simulink library "Libs_second"  (R2023b)
settings: Solver=VariableStepAuto  StartTime=0.0  StopTime=10.0  RelTol=1e-3
libraries: $bdroot x3, simulink x1
(part 1 of 2)
settings Model: Creator=wai484  LastModifiedBy=wai484
settings SolverCC: AlgebraicLoopSolver=TrustRegion
settings DataIOCC: ReturnWorkspaceOutputs=off
settings DebuggingCC: UnconnectedInputMsg=warning  UnconnectedOutputMsg=warning  UnconnectedLineMsg=warning  ArithmeticOperatorsInVariantConditions=warning
settings ModelReferenceCC: EnableRefExpFcnMdlSchedulingChecks=on
settings SFSimCC: SimUseLocalCustomCode=off  CustomCodeUndefinedFunction=UseInterfaceOnly
settings RTWCC: RTWUseLocalCustomCode=off
settings CodeAppCC: StateflowObjectComments=on

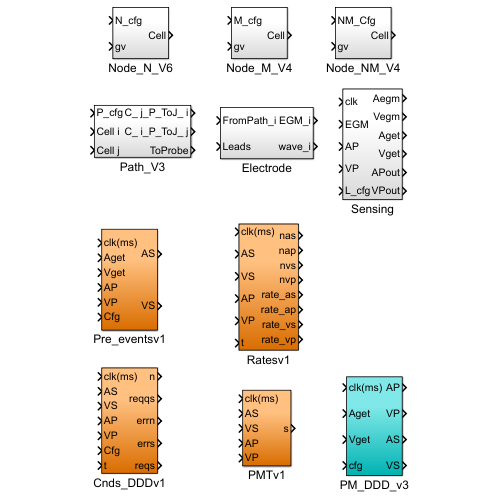
[thumbnail: Simulink's stored preview of the top-level diagram]
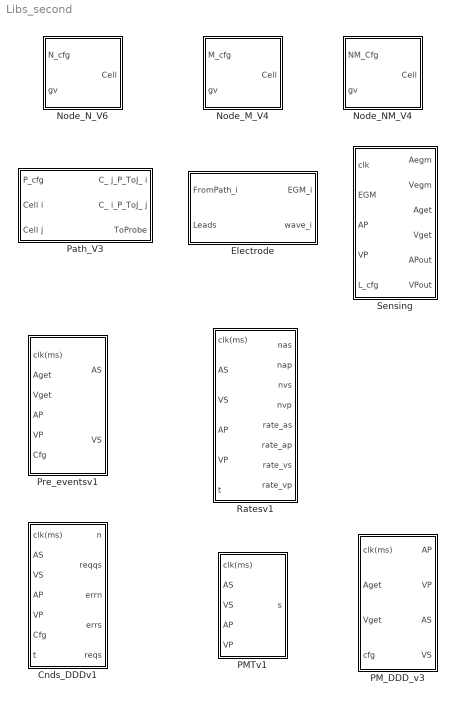
== system Libs_second ==
  Cnds_DDDv1 : Subsystem
  Electrode : Subsystem
  Node_M_V4 : Subsystem
  Node_NM_V4 : Subsystem
  Node_N_V6 : Subsystem
  PMTv1 : Subsystem
  PM_DDD_v3 : Subsystem
  Path_V3 : Subsystem
  Pre_eventsv1 : Subsystem
  Ratesv1 : Subsystem
  Sensing : Subsystem

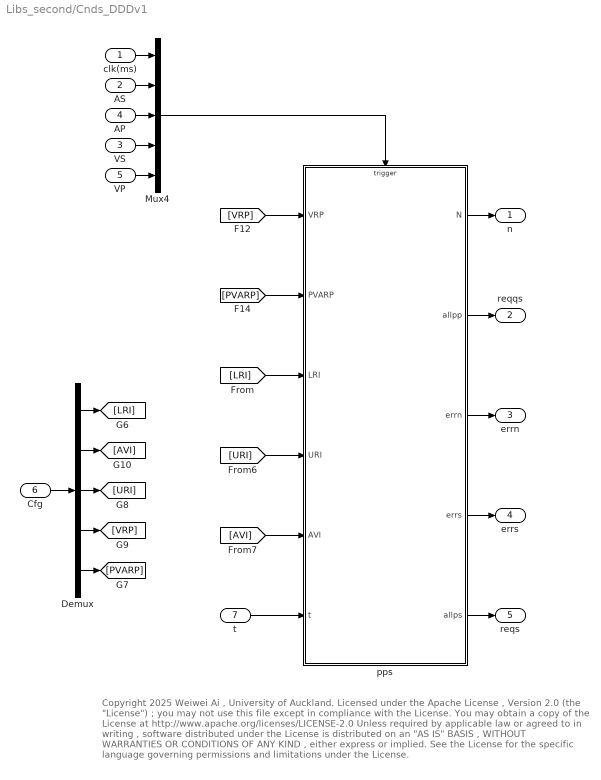
== system Libs_second/Cnds_DDDv1 ==
  note: Copyright 2025 Weiwei Ai , University of Auckland.
      | Licensed under the Apache License , Version 2.0 (the "License") ;
      | you may not use this file except in compliance with the License.
      | You may obtain a copy of the License at
      | http://www.apache.org/licenses/LICENSE-2.0
      | Unless required by applicable law or agreed to in writing , software
      | distributed under the License is distributed on an "AS IS" BASIS ,
      | WITHOUT WARRANTIES OR CONDITIONS OF ANY KIND , either express or implied.
      | See the License for the specific language governing permissions and
      | limitations under the License.
  clk(ms) : Inport
  AS : Inport  Port=2
  VS : Inport  Port=3
  AP : Inport  Port=4
  VP : Inport  Port=5
  Cfg : Inport  Port=6
  t : Inport  Port=7
  Demux : Demux  Outputs=5
  Mux4 : Mux  Inputs=5
  pps : Stateflow chart  TreatAsAtomicUnit=on
  n : Outport
  reqqs : Outport  Port=2
  errn : Outport  Port=3
  errs : Outport  Port=4
  reqs : Outport  Port=5
  wires:
  t/1 -> pps/6(t)
  pps/5(allps) -> reqs/1
  Demux/5 -> [PVARP]
  Demux/4 -> [VRP]
  Demux/3 -> [URI]
  Demux/2 -> [AVI]
  Demux/1 -> [LRI]
  pps/4(errs) -> errs/1
  pps/3(errn) -> errn/1
  pps/2(allpp) -> reqqs/1
  pps/1(N) -> n/1
  [VRP] -> pps/1(VRP)
  [PVARP] -> pps/2(PVARP)
  [LRI] -> pps/3(LRI)
  [AVI] -> pps/5(AVI)
  [URI] -> pps/4(URI)
  Cfg/1 -> Demux/1
  clk(ms)/1 -> Mux4/1
  AS/1 -> Mux4/2
  VP/1 -> Mux4/5
  Mux4/1 -> pps/Trigger
  AP/1 -> Mux4/3
  VS/1 -> Mux4/4

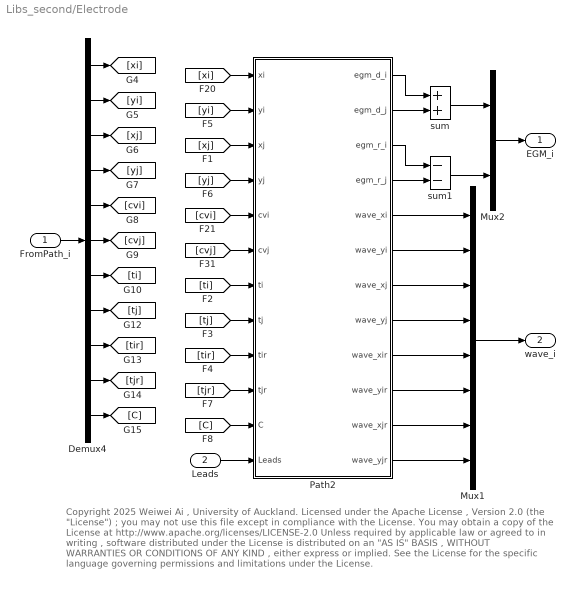
== system Libs_second/Electrode ==
  note: Copyright 2025 Weiwei Ai , University of Auckland.
      | Licensed under the Apache License , Version 2.0 (the "License") ;
      | you may not use this file except in compliance with the License.
      | You may obtain a copy of the License at
      | http://www.apache.org/licenses/LICENSE-2.0
      | Unless required by applicable law or agreed to in writing , software
      | distributed under the License is distributed on an "AS IS" BASIS ,
      | WITHOUT WARRANTIES OR CONDITIONS OF ANY KIND , either express or implied.
      | See the License for the specific language governing permissions and
      | limitations under the License.
  FromPath_i : Inport
  Leads : Inport  Port=2
  Demux4 : Demux  Outputs=11
  Mux1 : Mux  Inputs=8
  Mux2 : Mux  Inputs=2
  Path2 : Stateflow chart  TreatAsAtomicUnit=on
  sum : Sum
  sum1 : Sum  Inputs=--
  EGM_i : Outport
  wave_i : Outport  Port=2
  wires:
  Mux2/1 -> EGM_i/1
  [xi] -> Path2/1(xi)
  [xj] -> Path2/3(xj)
  [yi] -> Path2/2(yi)
  [yj] -> Path2/4(yj)
  [cvi] -> Path2/5(cvi)
  [cvj] -> Path2/6(cvj)
  FromPath_i/1 -> Demux4/1
  Demux4/1 -> [xi]
  Demux4/2 -> [yi]
  Demux4/3 -> [xj]
  Demux4/4 -> [yj]
  Demux4/5 -> [cvi]
  Demux4/6 -> [cvj]
  Demux4/7 -> [ti]
  Demux4/8 -> [tj]
  Demux4/9 -> [tir]
  Demux4/10 -> [tjr]
  Demux4/11 -> [C]
  Path2/5(wave_xi) -> Mux1/1
  Path2/6(wave_yi) -> Mux1/2
  Path2/7(wave_xj) -> Mux1/3
  Path2/8(wave_yj) -> Mux1/4
  [C] -> Path2/11(C)
  [tjr] -> Path2/10(tjr)
  [tir] -> Path2/9(tir)
  [tj] -> Path2/8(tj)
  [ti] -> Path2/7(ti)
  Leads/1 -> Path2/12(Leads)
  Path2/9(wave_xir) -> Mux1/5
  Path2/10(wave_yir) -> Mux1/6
  Path2/11(wave_xjr) -> Mux1/7
  Path2/12(wave_yjr) -> Mux1/8
  Mux1/1 -> wave_i/1
  sum/1 -> Mux2/1
  Path2/1(egm_d_i) -> sum/1
  Path2/2(egm_d_j) -> sum/2
  sum1/1 -> Mux2/2
  Path2/3(egm_r_i) -> sum1/1
  Path2/4(egm_r_j) -> sum1/2

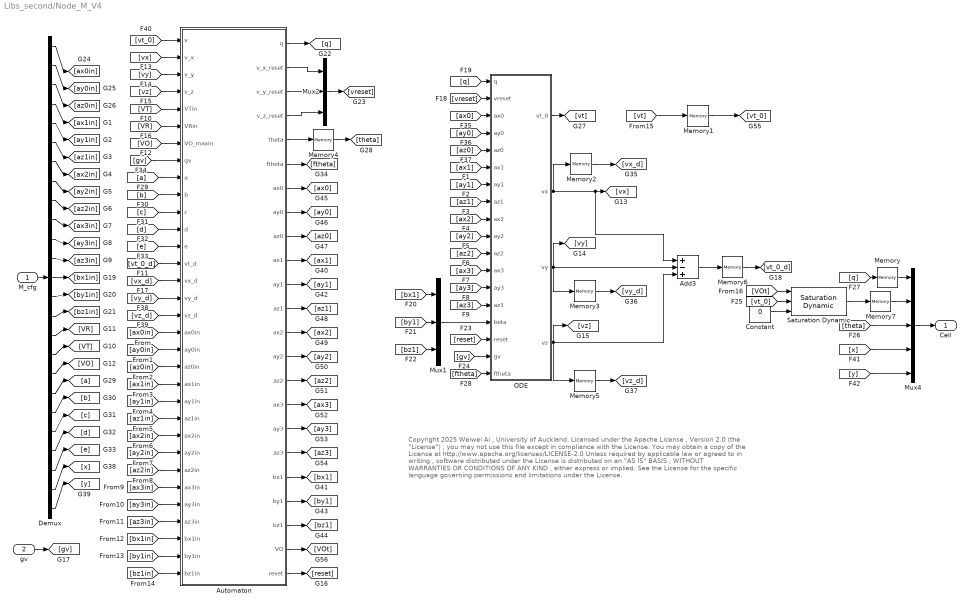
== system Libs_second/Node_M_V4 ==
  note: Copyright 2025 Weiwei Ai , University of Auckland.
      | Licensed under the Apache License , Version 2.0 (the "License") ;
      | you may not use this file except in compliance with the License.
      | You may obtain a copy of the License at
      | http://www.apache.org/licenses/LICENSE-2.0
      | Unless required by applicable law or agreed to in writing , software
      | distributed under the License is distributed on an "AS IS" BASIS ,
      | WITHOUT WARRANTIES OR CONDITIONS OF ANY KIND , either express or implied.
      | See the License for the specific language governing permissions and
      | limitations under the License.
  M_cfg : Inport
  gv : Inport  Port=2
  Add3 : Sum  Inputs=+-+
  Automaton : Stateflow chart  TreatAsAtomicUnit=on
  Constant : Constant  Value=0
  Demux : Demux  Outputs=25
  Memory : Memory
  Memory{1..3,5..7} (6 alike) : Memory  InheritSampleTime=on  LinearizeAsDelay=on
  Memory4 : Memory
  Mux1 : Mux  Inputs=3
  Mux2 : Mux  Inputs=3
  Mux4 : Mux  Inputs=5
  ODE : Subsystem
  Saturation Dynamic : simulink/Discontinuities/Saturation Dynamic  OutMin=[]  OutMax=[]  OutDataTypeStr=Inherit: Same as second input  OutDataType=fixdt(1, 16)  OutScaling=2^-10  DoSatur=off
  Cell : Outport
  wires:
  M_cfg/1 -> Demux/1
  Automaton/2(v_x_reset) -> Mux2/1
  Automaton/3(v_y_reset) -> Mux2/2
  Automaton/4(v_z_reset) -> Mux2/3
  Mux4/1 -> Cell/1
  Demux/1 -> [ax0in]
  [ax0] -> ODE/3(ax0)
  Demux/2 -> [ay0in]
  [ay0] -> ODE/4(ay0)
  [az0] -> ODE/5(az0)
  Demux/3 -> [az0in]
  [ay1] -> ODE/7(ay1)
  [az1] -> ODE/8(az1)
  [ax2] -> ODE/9(ax2)
  [ay2] -> ODE/10(ay2)
  [az2] -> ODE/11(az2)
  [ax3] -> ODE/12(ax3)
  [ay3] -> ODE/13(ay3)
  [az3] -> ODE/14(az3)
  Demux/4 -> [ax1in]
  Demux/5 -> [ay1in]
  Demux/6 -> [az1in]
  Demux/7 -> [ax2in]
  Demux/8 -> [ay2in]
  Demux/9 -> [az2in]
  Demux/10 -> [ax3in]
  Demux/11 -> [ay3in]
  Demux/12 -> [az3in]
  [VT] -> Automaton/5(VTin)
  [VR] -> Automaton/6(VRin)
  Demux/18 -> [VO]
  [VO] -> Automaton/7(VO_maxin)
  ODE/2(vx) -> Memory2/1, Add3/1, [vx]
  ODE/3(vy) -> Add3/2, Memory3/1, [vy]
  ODE/4(vz) -> Add3/3, Memory5/1, [vz]
  [vx] -> Automaton/2(v_x)
  [vy] -> Automaton/3(v_y)
  [vz] -> Automaton/4(v_z)
  [bx1] -> Mux1/1
  [by1] -> Mux1/2
  [bz1] -> Mux1/3
  Mux1/1 -> ODE/15(beta)
  Demux/13 -> [bx1in]
  Demux/14 -> [by1in]
  Demux/15 -> [bz1in]
  Demux/16 -> [VR]
  Demux/17 -> [VT]
  Automaton/23(reset) -> [reset]
  [reset] -> ODE/16(reset)
  [gv] -> ODE/17(gv)
  Mux2/1 -> [vreset]
  [vreset] -> ODE/2(vreset)
  Automaton/1(q) -> [q]
  [q] -> ODE/1(q)
  ODE/1(vt_0) -> [vt]
  Memory/1 -> Mux4/1
  [q] -> Memory/1
  [theta] -> Mux4/3
  Demux/19 -> [a]
  Demux/20 -> [b]
  Demux/21 -> [c]
  Demux/22 -> [d]
  Demux/23 -> [e]
  [ax1] -> ODE/6(ax1)
  Memory4/1 -> [theta]
  [ftheta] -> ODE/18(ftheta)
  [a] -> Automaton/9(a)
  [b] -> Automaton/10(b)
  [c] -> Automaton/11(c)
  [d] -> Automaton/12(d)
  [e] -> Automaton/13(e)
  Automaton/5(theta) -> Memory4/1
  Automaton/6(ftheta) -> [ftheta]
  Memory2/1 -> [vx_d]
  Memory3/1 -> [vy_d]
  Memory5/1 -> [vz_d]
  [vt_0_d] -> Automaton/14(vt_d)
  [vx_d] -> Automaton/15(vx_d)
  [vy_d] -> Automaton/16(vy_d)
  [vz_d] -> Automaton/17(vz_d)
  [vt_0] -> Automaton/1(v)
  Demux/24 -> [x]
  Demux/25 -> [y]
  [x] -> Mux4/4
  [y] -> Mux4/5
  gv/1 -> [gv]
  [gv] -> Automaton/8(gv)
  Automaton/21(bz1) -> [bz1]
  Automaton/20(by1) -> [by1]
  Automaton/19(bx1) -> [bx1]
  Automaton/18(az3) -> [az3]
  Automaton/7(ax0) -> [ax0]
  Automaton/8(ay0) -> [ay0]
  Automaton/9(az0) -> [az0]
  Automaton/10(ax1) -> [ax1]
  Automaton/11(ay1) -> [ay1]
  Automaton/12(az1) -> [az1]
  Automaton/13(ax2) -> [ax2]
  Automaton/14(ay2) -> [ay2]
  Automaton/16(ax3) -> [ax3]
  Automaton/15(az2) -> [az2]
  [ax0in] -> Automaton/18(ax0in)
  [ay0in] -> Automaton/19(ay0in)
  [az0in] -> Automaton/20(az0in)
  [ax1in] -> Automaton/21(ax1in)
  [ay1in] -> Automaton/22(ay1in)
  [az1in] -> Automaton/23(az1in)
  [az2in] -> Automaton/26(az2in)
  [ax2in] -> Automaton/24(ax2in)
  [ay2in] -> Automaton/25(ay2in)
  Automaton/17(ay3) -> [ay3]
  [az3in] -> Automaton/29(az3in)
  [ay3in] -> Automaton/28(ay3in)
  [ax3in] -> Automaton/27(ax3in)
  [bz1in] -> Automaton/32(bz1in)
  [bx1in] -> Automaton/30(bx1in)
  [by1in] -> Automaton/31(by1in)
  Automaton/22(VO) -> [VOt]
  [vt] -> Memory1/1
  Memory1/1 -> [vt_0]
  Memory6/1 -> [vt_0_d]
  Add3/1 -> Memory6/1
  [vt_0] -> Saturation Dynamic/2
  [VOt] -> Saturation Dynamic/1
  Constant/1 -> Saturation Dynamic/3
  Memory7/1 -> Mux4/2
  Saturation Dynamic/1 -> Memory7/1

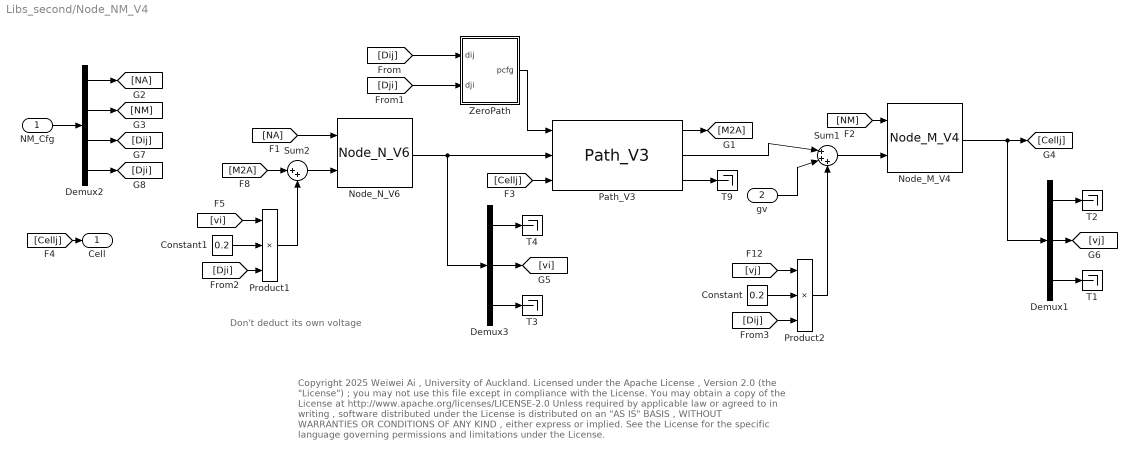
== system Libs_second/Node_NM_V4 ==
  note: Don't deduct its own voltage
  note: Copyright 2025 Weiwei Ai , University of Auckland.
      | Licensed under the Apache License , Version 2.0 (the "License") ;
      | you may not use this file except in compliance with the License.
      | You may obtain a copy of the License at
      | http://www.apache.org/licenses/LICENSE-2.0
      | Unless required by applicable law or agreed to in writing , software
      | distributed under the License is distributed on an "AS IS" BASIS ,
      | WITHOUT WARRANTIES OR CONDITIONS OF ANY KIND , either express or implied.
      | See the License for the specific language governing permissions and
      | limitations under the License.
  NM_Cfg : Inport
  gv : Inport  Port=2
  Constant : Constant  Value=0.2
  Constant1 : Constant  Value=0.2
  Demux1 : Demux  Outputs=[1,1,3]
  Demux2 : Demux  Outputs=[23,25,1,1]
  Demux3 : Demux  Outputs=[1,1,3]
  Node_M_V4 : $bdroot/Node_M_V4  SystemSampleTime=-1  VariantActivationTime=update diagram  AllowFlexibleInterface=on  Latency=0  AutoFrameSizeCalculation=off
  Node_N_V6 : $bdroot/Node_N_V6  SystemSampleTime=-1  VariantActivationTime=update diagram  AllowFlexibleInterface=on  Latency=0  AutoFrameSizeCalculation=off
  Path_V3 : $bdroot/Path_V3  SystemSampleTime=-1  VariantActivationTime=update diagram  AllowFlexibleInterface=on  Latency=0  AutoFrameSizeCalculation=off
  Product1 : Product  Inputs=***
  Product2 : Product  Inputs=***
  Sum1 : Sum  Inputs=|+++
  Sum2 : Sum  Inputs=|++
  T{1..4,9} (5 alike) : Terminator
  ZeroPath : MATLAB Function  TreatAsAtomicUnit=on
  Cell : Outport
  wires:
  NM_Cfg/1 -> Demux2/1
  Path_V3/3 -> T9/1
  Demux2/1 -> [NA]
  Demux2/2 -> [NM]
  [NA] -> Node_N_V6/1
  [NM] -> Node_M_V4/1
  Path_V3/1 -> [M2A]
  Node_M_V4/1 -> Demux1/1, [Cellj]
  [Cellj] -> Path_V3/3
  [Cellj] -> Cell/1
  ZeroPath/1(pcfg) -> Path_V3/1
  Path_V3/2 -> Sum1/1
  Sum1/1 -> Node_M_V4/2
  Demux1/3 -> T1/1
  Demux1/1 -> T2/1
  Node_N_V6/1 -> Path_V3/2, Demux3/1
  Demux3/3 -> T3/1
  Demux3/1 -> T4/1
  Demux3/2 -> [vi]
  Demux1/2 -> [vj]
  Constant/1 -> Product2/2
  [vj] -> Product2/1
  Product2/1 -> Sum1/3
  gv/1 -> Sum1/2
  [M2A] -> Sum2/1
  Sum2/1 -> Node_N_V6/2
  Constant1/1 -> Product1/2
  [vi] -> Product1/1
  Product1/1 -> Sum2/2
  Demux2/3 -> [Dij]
  Demux2/4 -> [Dji]
  [Dij] -> ZeroPath/1(dij)
  [Dji] -> ZeroPath/2(dji)
  [Dji] -> Product1/3
  [Dij] -> Product2/3

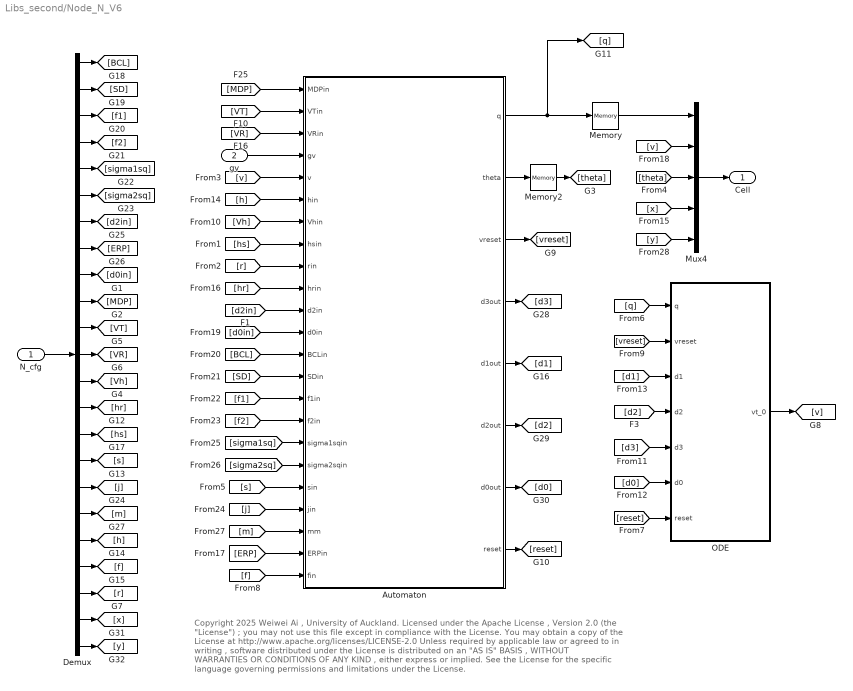
== system Libs_second/Node_N_V6 ==
  note: Copyright 2025 Weiwei Ai , University of Auckland.
      | Licensed under the Apache License , Version 2.0 (the "License") ;
      | you may not use this file except in compliance with the License.
      | You may obtain a copy of the License at
      | http://www.apache.org/licenses/LICENSE-2.0
      | Unless required by applicable law or agreed to in writing , software
      | distributed under the License is distributed on an "AS IS" BASIS ,
      | WITHOUT WARRANTIES OR CONDITIONS OF ANY KIND , either express or implied.
      | See the License for the specific language governing permissions and
      | limitations under the License.
  N_cfg : Inport
  gv : Inport  Port=2
  Automaton : Stateflow chart  TreatAsAtomicUnit=on
  Demux : Demux  Outputs=23
  Memory : Memory
  Memory2 : Memory
  Mux4 : Mux  Inputs=5
  ODE : Subsystem
  Cell : Outport
  wires:
  N_cfg/1 -> Demux/1
  Automaton/1(q) -> Memory/1, [q]
  Mux4/1 -> Cell/1
  Memory/1 -> Mux4/1
  [VR] -> Automaton/3(VRin)
  [VT] -> Automaton/2(VTin)
  [MDP] -> Automaton/1(MDPin)
  [r] -> Automaton/9(rin)
  [d1] -> ODE/3(d1)
  [d2] -> ODE/4(d2)
  [d3] -> ODE/5(d3)
  [d0] -> ODE/6(d0)
  [v] -> Automaton/5(v)
  ODE/1(vt_0) -> [v]
  Automaton/3(vreset) -> [vreset]
  Automaton/8(reset) -> [reset]
  [q] -> ODE/1(q)
  [reset] -> ODE/7(reset)
  [vreset] -> ODE/2(vreset)
  [Vh] -> Automaton/7(Vhin)
  [hs] -> Automaton/8(hsin)
  [h] -> Automaton/6(hin)
  [hr] -> Automaton/10(hrin)
  [v] -> Mux4/2
  [theta] -> Mux4/3
  Automaton/2(theta) -> Memory2/1
  Memory2/1 -> [theta]
  Automaton/5(d1out) -> [d1]
  [d2in] -> Automaton/11(d2in)
  [d0in] -> Automaton/12(d0in)
  [BCL] -> Automaton/13(BCLin)
  [SD] -> Automaton/14(SDin)
  [f1] -> Automaton/15(f1in)
  [f2] -> Automaton/16(f2in)
  [sigma1sq] -> Automaton/17(sigma1sqin)
  [sigma2sq] -> Automaton/18(sigma2sqin)
  Demux/1 -> [BCL]
  Demux/2 -> [SD]
  Demux/3 -> [f1]
  Demux/4 -> [f2]
  Demux/5 -> [sigma1sq]
  Demux/6 -> [sigma2sq]
  Demux/7 -> [d2in]
  Demux/8 -> [ERP]
  Demux/9 -> [d0in]
  Demux/10 -> [MDP]
  Demux/11 -> [VT]
  Demux/12 -> [VR]
  Demux/16 -> [s]
  Demux/15 -> [hs]
  Demux/14 -> [hr]
  Demux/13 -> [Vh]
  [s] -> Automaton/19(sin)
  [j] -> Automaton/20(jin)
  Demux/17 -> [j]
  Demux/21 -> [r]
  Demux/20 -> [f]
  Demux/19 -> [h]
  Demux/18 -> [m]
  [m] -> Automaton/21(mm)
  [ERP] -> Automaton/22(ERPin)
  Automaton/4(d3out) -> [d3]
  [f] -> Automaton/23(fin)
  Automaton/6(d2out) -> [d2]
  Automaton/7(d0out) -> [d0]
  Demux/22 -> [x]
  Demux/23 -> [y]
  [x] -> Mux4/4
  [y] -> Mux4/5
  gv/1 -> Automaton/4(gv)

== system Libs_second/PMTv1 ==
  note: Adapta ADDRS1 pacemaker (Medtronic)
  note: Copyright 2025 Weiwei Ai , University of Auckland.
      | Licensed under the Apache License , Version 2.0 (the "License") ;
      | you may not use this file except in compliance with the License.
      | You may obtain a copy of the License at
      | http://www.apache.org/licenses/LICENSE-2.0
      | Unless required by applicable law or agreed to in writing , software
      | distributed under the License is distributed on an "AS IS" BASIS ,
      | WITHOUT WARRANTIES OR CONDITIONS OF ANY KIND , either express or implied.
      | See the License for the specific language governing permissions and
      | limitations under the License.
  clk(ms) : Inport
  AS : Inport  Port=2
  VS : Inport  Port=3
  AP : Inport  Port=4
  VP : Inport  Port=5
  Mux4 : Mux  Inputs=5
  PMT detection : Stateflow chart  TreatAsAtomicUnit=on
  s : Outport
  wires:
  PMT detection/1(s) -> s/1
  clk(ms)/1 -> Mux4/1
  AS/1 -> Mux4/2
  VS/1 -> Mux4/3
  AP/1 -> Mux4/4
  VP/1 -> Mux4/5
  Mux4/1 -> PMT detection/Trigger

== system Libs_second/PM_DDD_v3 ==
  note: Copyright 2025 Weiwei Ai , University of Auckland.
      | Licensed under the Apache License , Version 2.0 (the "License") ;
      | you may not use this file except in compliance with the License.
      | You may obtain a copy of the License at
      | http://www.apache.org/licenses/LICENSE-2.0
      | Unless required by applicable law or agreed to in writing , software
      | distributed under the License is distributed on an "AS IS" BASIS ,
      | WITHOUT WARRANTIES OR CONDITIONS OF ANY KIND , either express or implied.
      | See the License for the specific language governing permissions and
      | limitations under the License.
  clk(ms) : Inport
  Aget : Inport  Port=2
  Vget : Inport  Port=3
  cfg : Inport  Port=4
  DDD : Stateflow chart  TreatAsAtomicUnit=on
  Demux : Demux  Outputs=5
  Memory : Memory
  Memory1 : Memory
  Memory7 : Memory
  Mux{1..4} (4 alike) : Mux  Inputs=2
  conv : DataTypeConversion  SaturateOnIntegerOverflow=off  RndMeth=Floor
  pul : Stateflow chart  TreatAsAtomicUnit=on
  pul1 : Stateflow chart  TreatAsAtomicUnit=on
  pul2 : Stateflow chart  TreatAsAtomicUnit=on
  pul3 : Stateflow chart  TreatAsAtomicUnit=on
  AP : Outport
  VP : Outport  Port=2
  AS : Outport  Port=3
  VS : Outport  Port=4
  wires:
  Memory7/1 -> Demux/1
  cfg/1 -> Memory7/1
  DDD/2(VP) -> Memory1/1
  Memory/1 -> Mux3/2
  DDD/1(AP) -> Memory/1
  Demux/5 -> DDD/5(PVARPd)
  Demux/4 -> DDD/4(VRPd)
  Demux/3 -> DDD/3(URId)
  Demux/2 -> DDD/2(AVId)
  Demux/1 -> DDD/1(LRId)
  clk(ms)/1 -> conv/1, DDD/Trigger
  Aget/1 -> DDD/6(AinB)
  Vget/1 -> DDD/7(VinB)
  pul/1(eve) -> AP/1
  pul3/1(eve) -> VS/1
  pul1/1(eve) -> VP/1
  pul2/1(eve) -> AS/1
  [clkms] -> Mux4/1, Mux2/1, Mux1/1, Mux3/1
  Mux3/1 -> pul/Trigger
  Memory1/1 -> Mux1/2
  Mux1/1 -> pul1/Trigger
  Mux2/1 -> pul2/Trigger
  Mux4/1 -> pul3/Trigger
  DDD/4(VS) -> Mux4/2
  DDD/3(AS) -> Mux2/2
  conv/1 -> [clkms]

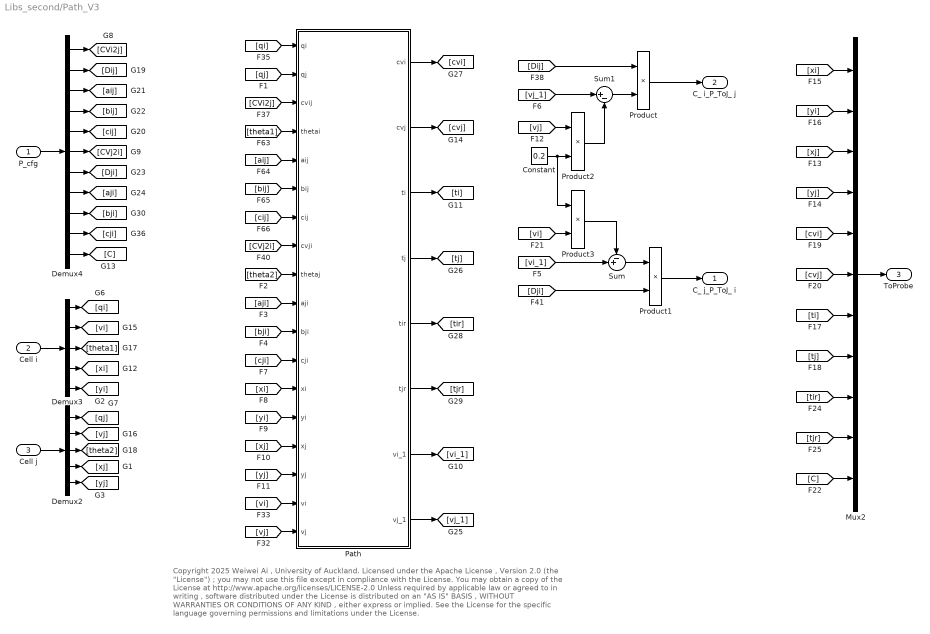
== system Libs_second/Path_V3 ==
  note: Copyright 2025 Weiwei Ai , University of Auckland.
      | Licensed under the Apache License , Version 2.0 (the "License") ;
      | you may not use this file except in compliance with the License.
      | You may obtain a copy of the License at
      | http://www.apache.org/licenses/LICENSE-2.0
      | Unless required by applicable law or agreed to in writing , software
      | distributed under the License is distributed on an "AS IS" BASIS ,
      | WITHOUT WARRANTIES OR CONDITIONS OF ANY KIND , either express or implied.
      | See the License for the specific language governing permissions and
      | limitations under the License.
  P_cfg : Inport
  Cell i : Inport  Port=2
  Cell j : Inport  Port=3
  Constant : Constant  Value=0.2
  Demux2 : Demux  Outputs=5
  Demux3 : Demux  Outputs=5
  Demux4 : Demux  Outputs=11
  Mux2 : Mux  Inputs=11
  Path : Stateflow chart  TreatAsAtomicUnit=on
  Product{,1..3} (4 alike) : Product  Inputs=**
  Sum : Sum  Inputs=-+|
  Sum1 : Sum  Inputs=|+-
  C_ j_P_ToJ_ i : Outport
  C_ i_P_ToJ_ j : Outport  Port=2
  ToProbe : Outport  Port=3
  wires:
  Cell i/1 -> Demux3/1
  Cell j/1 -> Demux2/1
  P_cfg/1 -> Demux4/1
  Product/1 -> C_ i_P_ToJ_ j/1
  Product1/1 -> C_ j_P_ToJ_ i/1
  Demux3/1 -> [qi]
  [qi] -> Path/1(qi)
  Demux2/1 -> [qj]
  Demux3/4 -> [xi]
  Demux3/5 -> [yi]
  Demux2/4 -> [xj]
  Demux2/5 -> [yj]
  Demux3/2 -> [vi]
  [vi] -> Path/17(vi)
  Demux2/2 -> [vj]
  [vj] -> Path/18(vj)
  Demux3/3 -> [theta1]
  Demux2/3 -> [theta2]
  [Dij] -> Product/1
  [theta1] -> Path/4(thetai)
  [aij] -> Path/5(aij)
  [bij] -> Path/6(bij)
  [cij] -> Path/7(cij)
  Demux4/2 -> [Dij]
  Demux4/3 -> [aij]
  Demux4/4 -> [bij]
  Demux4/5 -> [cij]
  Demux4/1 -> [CVi2j]
  [xi] -> Path/13(xi)
  [yi] -> Path/14(yi)
  [xj] -> Path/15(xj)
  [yj] -> Path/16(yj)
  [CVi2j] -> Path/3(cvij)
  Demux4/11 -> [C]
  Demux4/10 -> [cji]
  Demux4/9 -> [bji]
  Demux4/8 -> [aji]
  Demux4/7 -> [Dji]
  Demux4/6 -> [CVj2i]
  [cji] -> Path/12(cji)
  [bji] -> Path/11(bji)
  [aji] -> Path/10(aji)
  [theta2] -> Path/9(thetaj)
  [CVj2i] -> Path/8(cvji)
  [qj] -> Path/2(qj)
  Path/8(vj_1) -> [vj_1]
  Path/7(vi_1) -> [vi_1]
  Path/1(cvi) -> [cvi]
  Path/2(cvj) -> [cvj]
  Path/3(ti) -> [ti]
  Path/4(tj) -> [tj]
  Path/5(tir) -> [tir]
  Path/6(tjr) -> [tjr]
  [xi] -> Mux2/1
  [yi] -> Mux2/2
  [xj] -> Mux2/3
  [yj] -> Mux2/4
  [cvi] -> Mux2/5
  [tir] -> Mux2/9
  [cvj] -> Mux2/6
  [ti] -> Mux2/7
  [tj] -> Mux2/8
  [tjr] -> Mux2/10
  [C] -> Mux2/11
  Mux2/1 -> ToProbe/1
  [vj_1] -> Sum1/1
  Sum1/1 -> Product/2
  [vj] -> Product2/1
  Product2/1 -> Sum1/2
  Constant/1 -> Product3/1, Product2/2
  Sum/1 -> Product1/1
  Product3/1 -> Sum/1
  [vi_1] -> Sum/2
  [Dji] -> Product1/2
  [vi] -> Product3/2

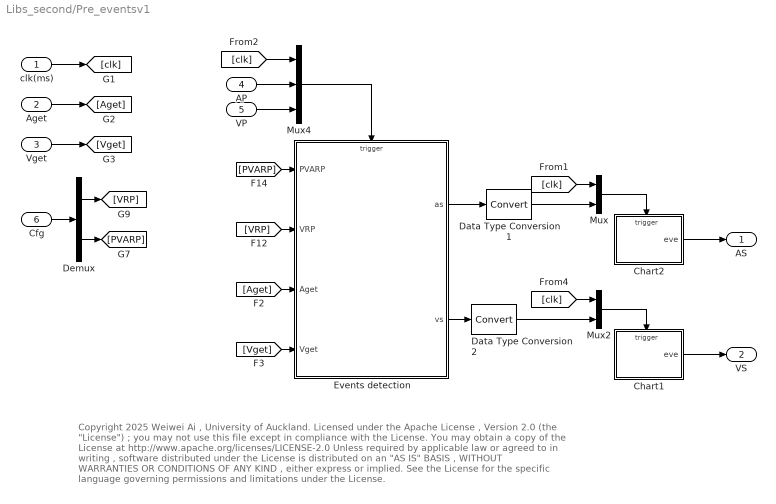
== system Libs_second/Pre_eventsv1 ==
  note: Copyright 2025 Weiwei Ai , University of Auckland.
      | Licensed under the Apache License , Version 2.0 (the "License") ;
      | you may not use this file except in compliance with the License.
      | You may obtain a copy of the License at
      | http://www.apache.org/licenses/LICENSE-2.0
      | Unless required by applicable law or agreed to in writing , software
      | distributed under the License is distributed on an "AS IS" BASIS ,
      | WITHOUT WARRANTIES OR CONDITIONS OF ANY KIND , either express or implied.
      | See the License for the specific language governing permissions and
      | limitations under the License.
  clk(ms) : Inport
  Aget : Inport  Port=2
  Vget : Inport  Port=3
  AP : Inport  Port=4
  VP : Inport  Port=5
  Cfg : Inport  Port=6
  Chart1 : Stateflow chart  TreatAsAtomicUnit=on
  Chart2 : Stateflow chart  TreatAsAtomicUnit=on
  Data Type Conversion1 : DataTypeConversion  SaturateOnIntegerOverflow=off  RndMeth=Floor
  Data Type Conversion2 : DataTypeConversion  SaturateOnIntegerOverflow=off  RndMeth=Floor
  Demux : Demux  Outputs=2
  Events detection : Stateflow chart  TreatAsAtomicUnit=on
  Mux : Mux  Inputs=2
  Mux2 : Mux  Inputs=2
  Mux4 : Mux  Inputs=3
  AS : Outport
  VS : Outport  Port=2
  wires:
  clk(ms)/1 -> [clk]
  Events detection/2(vs) -> Data Type Conversion2/1
  Chart1/1(eve) -> VS/1
  [clk] -> Mux2/1
  Mux2/1 -> Chart1/Trigger
  [clk] -> Mux/1
  Events detection/1(as) -> Data Type Conversion1/1
  Chart2/1(eve) -> AS/1
  Mux/1 -> Chart2/Trigger
  [Vget] -> Events detection/4(Vget)
  [Aget] -> Events detection/3(Aget)
  Vget/1 -> [Vget]
  Aget/1 -> [Aget]
  [VRP] -> Events detection/2(VRP)
  AP/1 -> Mux4/2
  Cfg/1 -> Demux/1
  VP/1 -> Mux4/3
  [clk] -> Mux4/1
  [PVARP] -> Events detection/1(PVARP)
  Mux4/1 -> Events detection/Trigger
  Demux/1 -> [VRP]
  Demux/2 -> [PVARP]
  Data Type Conversion1/1 -> Mux/2
  Data Type Conversion2/1 -> Mux2/2

== system Libs_second/Ratesv1 ==
  note: Copyright 2025 Weiwei Ai , University of Auckland.
      | Licensed under the Apache License , Version 2.0 (the "License") ;
      | you may not use this file except in compliance with the License.
      | You may obtain a copy of the License at
      | http://www.apache.org/licenses/LICENSE-2.0
      | Unless required by applicable law or agreed to in writing , software
      | distributed under the License is distributed on an "AS IS" BASIS ,
      | WITHOUT WARRANTIES OR CONDITIONS OF ANY KIND , either express or implied.
      | See the License for the specific language governing permissions and
      | limitations under the License.
  clk(ms) : Inport
  AS : Inport  Port=2
  VS : Inport  Port=3
  AP : Inport  Port=4
  VP : Inport  Port=5
  t : Inport  Port=6
  Mux4 : Mux  Inputs=5
  rates : Stateflow chart  TreatAsAtomicUnit=on
  nas : Outport
  nap : Outport  Port=2
  nvs : Outport  Port=3
  nvp : Outport  Port=4
  rate_as : Outport  Port=5
  rate_ap : Outport  Port=6
  rate_vs : Outport  Port=7
  rate_vp : Outport  Port=8
  wires:
  clk(ms)/1 -> Mux4/1
  AS/1 -> Mux4/2
  VS/1 -> Mux4/3
  AP/1 -> Mux4/4
  VP/1 -> Mux4/5
  Mux4/1 -> rates/Trigger
  t/1 -> rates/1(t)
  rates/1(nas) -> nas/1
  rates/2(nap) -> nap/1
  rates/3(nvs) -> nvs/1
  rates/4(nvp) -> nvp/1
  rates/5(rate_as) -> rate_as/1
  rates/6(rate_ap) -> rate_ap/1
  rates/7(rate_vs) -> rate_vs/1
  rates/8(rate_vp) -> rate_vp/1

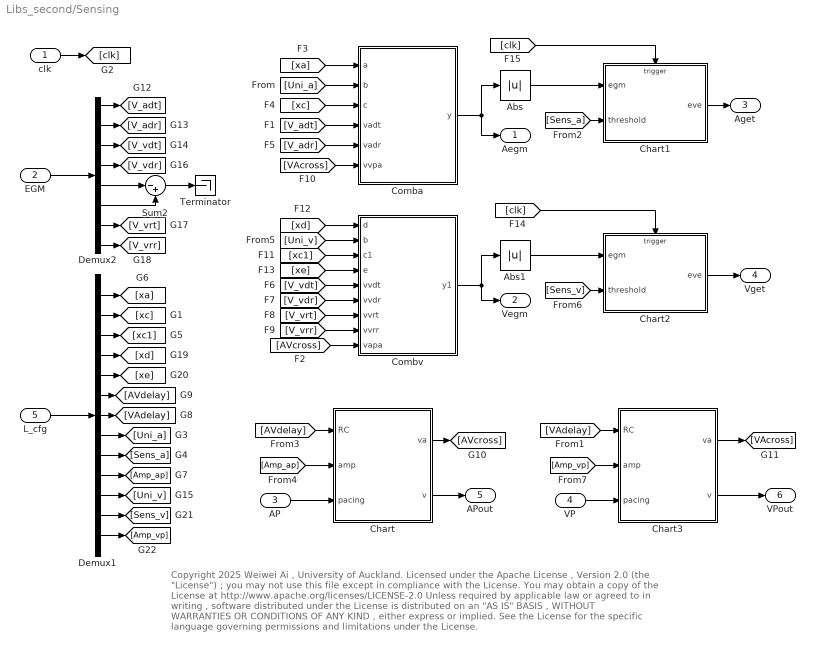
== system Libs_second/Sensing ==
  note: Copyright 2025 Weiwei Ai , University of Auckland.
      | Licensed under the Apache License , Version 2.0 (the "License") ;
      | you may not use this file except in compliance with the License.
      | You may obtain a copy of the License at
      | http://www.apache.org/licenses/LICENSE-2.0
      | Unless required by applicable law or agreed to in writing , software
      | distributed under the License is distributed on an "AS IS" BASIS ,
      | WITHOUT WARRANTIES OR CONDITIONS OF ANY KIND , either express or implied.
      | See the License for the specific language governing permissions and
      | limitations under the License.
  clk : Inport
  EGM : Inport  Port=2
  AP : Inport  Port=3
  VP : Inport  Port=4
  L_cfg : Inport  Port=5
  Abs : Abs  SaturateOnIntegerOverflow=off
  Abs1 : Abs  SaturateOnIntegerOverflow=off
  Chart : Stateflow chart  TreatAsAtomicUnit=on
  Chart1 : Stateflow chart  TreatAsAtomicUnit=on
  Chart2 : Stateflow chart  TreatAsAtomicUnit=on
  Chart3 : Stateflow chart  TreatAsAtomicUnit=on
  Comba : MATLAB Function  TreatAsAtomicUnit=on
  Combv : MATLAB Function  TreatAsAtomicUnit=on
  Demux1 : Demux  Outputs=13
  Demux2 : Demux  Outputs=8
  Sum2 : Sum  Inputs=|-+
  Terminator : Terminator
  Aegm : Outport
  Vegm : Outport  Port=2
  Aget : Outport  Port=3
  Vget : Outport  Port=4
  APout : Outport  Port=5
  VPout : Outport  Port=6
  wires:
  EGM/1 -> Demux2/1
  L_cfg/1 -> Demux1/1
  Demux2/5 -> Sum2/1
  Demux2/6 -> Sum2/2
  Sum2/1 -> Terminator/1
  Comba/1(y) -> Aegm/1, Abs/1
  AP/1 -> Chart/3(pacing)
  [AVdelay] -> Chart/1(RC)
  VP/1 -> Chart3/3(pacing)
  Demux2/1 -> [V_adt]
  Demux2/2 -> [V_adr]
  Demux2/3 -> [V_vdt]
  Demux2/4 -> [V_vdr]
  Demux2/7 -> [V_vrt]
  Demux2/8 -> [V_vrr]
  [V_adt] -> Comba/4(vadt)
  [V_adr] -> Comba/5(vadr)
  [V_vdt] -> Combv/5(vvdt)
  [V_vdr] -> Combv/6(vvdr)
  [V_vrt] -> Combv/7(vvrt)
  [V_vrr] -> Combv/8(vvrr)
  [xa] -> Comba/1(a)
  [xc] -> Comba/3(c)
  [xd] -> Combv/1(d)
  Combv/1(y1) -> Abs1/1, Vegm/1
  [xc1] -> Combv/3(c1)
  [xe] -> Combv/4(e)
  [AVcross] -> Combv/9(vapa)
  [VAcross] -> Comba/6(vvpa)
  Chart/1(va) -> [AVcross]
  Chart/2(v) -> APout/1
  Chart3/1(va) -> [VAcross]
  Chart3/2(v) -> VPout/1
  [VAdelay] -> Chart3/1(RC)
  Chart1/1(eve) -> Aget/1
  Abs/1 -> Chart1/1(egm)
  clk/1 -> [clk]
  [clk] -> Chart1/Trigger
  Demux1/1 -> [xa]
  Demux1/2 -> [xc]
  Demux1/6 -> [AVdelay]
  Demux1/3 -> [xc1]
  Demux1/4 -> [xd]
  Demux1/5 -> [xe]
  Demux1/7 -> [VAdelay]
  Demux1/8 -> [Uni_a]
  Demux1/9 -> [Sens_a]
  Demux1/10 -> [Amp_ap]
  Demux1/11 -> [Uni_v]
  Demux1/12 -> [Sens_v]
  Demux1/13 -> [Amp_vp]
  [Uni_a] -> Comba/2(b)
  [Uni_v] -> Combv/2(b)
  [Sens_a] -> Chart1/2(threshold)
  [Amp_ap] -> Chart/2(amp)
  Chart2/1(eve) -> Vget/1
  Abs1/1 -> Chart2/1(egm)
  [clk] -> Chart2/Trigger
  [Sens_v] -> Chart2/2(threshold)
  [Amp_vp] -> Chart3/2(amp)

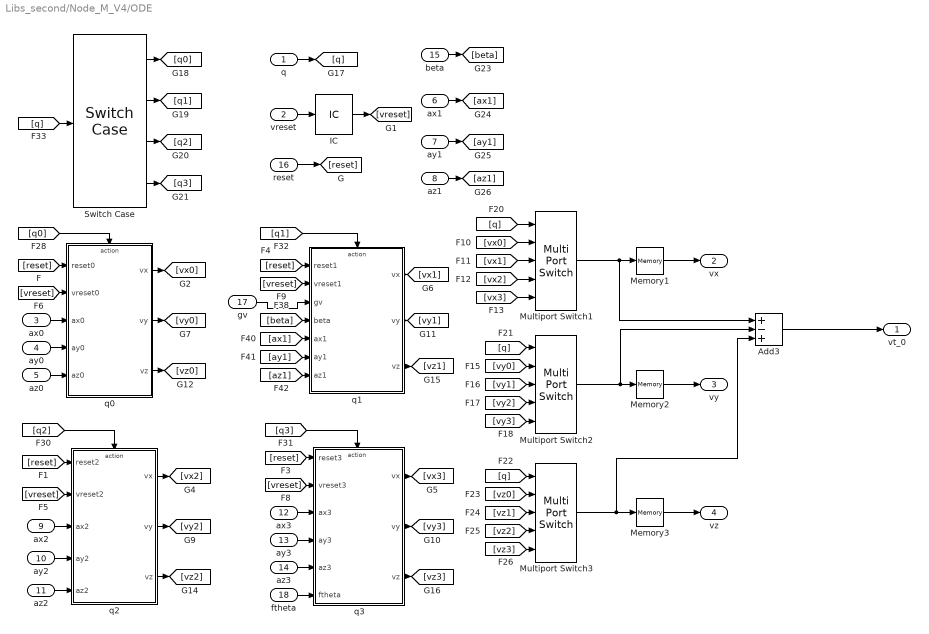
== system Libs_second/Node_M_V4/ODE ==
  q : Inport
  vreset : Inport  Port=2
  ax0 : Inport  Port=3
  ay0 : Inport  Port=4
  az0 : Inport  Port=5
  ax1 : Inport  Port=6
  ay1 : Inport  Port=7
  az1 : Inport  Port=8
  ax2 : Inport  Port=9
  ay2 : Inport  Port=10
  az2 : Inport  Port=11
  ax3 : Inport  Port=12
  ay3 : Inport  Port=13
  az3 : Inport  Port=14
  beta : Inport  Port=15
  reset : Inport  Port=16
  gv : Inport  Port=17
  ftheta : Inport  Port=18
  Add3 : Sum  Inputs=+-+
  IC : InitialCondition  Value=0
  Memory1 : Memory
  Memory2 : Memory
  Memory3 : Memory
  Multiport Switch1 : MultiPortSwitch  DataPortOrder=Zero-based contiguous  Inputs=4  zeroidx=on  SaturateOnIntegerOverflow=off  InputSameDT=off
  Multiport Switch2 : MultiPortSwitch  DataPortOrder=Zero-based contiguous  Inputs=4  zeroidx=on  SaturateOnIntegerOverflow=off  InputSameDT=off
  Multiport Switch3 : MultiPortSwitch  DataPortOrder=Zero-based contiguous  Inputs=4  zeroidx=on  SaturateOnIntegerOverflow=off  InputSameDT=off
  Switch Case : SwitchCase  CaseConditions={0,1,2,3}  ShowDefaultCase=off
  q0 : Subsystem  TreatAsAtomicUnit=on
  q1 : Subsystem  TreatAsAtomicUnit=on
  q2 : Subsystem  TreatAsAtomicUnit=on
  q3 : Subsystem  TreatAsAtomicUnit=on
  vt_0 : Outport
  vx : Outport  Port=2
  vy : Outport  Port=3
  vz : Outport  Port=4
  wires:
  gv/1 -> q1/3(gv)
  Multiport Switch2/1 -> Add3/2, Memory2/1
  Multiport Switch1/1 -> Add3/1, Memory1/1
  IC/1 -> [vreset]
  vreset/1 -> IC/1
  Memory3/1 -> vz/1
  Memory2/1 -> vy/1
  Memory1/1 -> vx/1
  ay3/1 -> q3/4(ay3)
  az2/1 -> q2/5(az2)
  ay2/1 -> q2/4(ay2)
  az0/1 -> q0/5(az0)
  ay0/1 -> q0/4(ay0)
  reset/1 -> [reset]
  ax0/1 -> q0/3(ax0)
  q/1 -> [q]
  ax2/1 -> q2/3(ax2)
  Add3/1 -> vt_0/1
  ax3/1 -> q3/3(ax3)
  ftheta/1 -> q3/6(ftheta)
  [reset] -> q0/1(reset0)
  [reset] -> q2/1(reset2)
  [reset] -> q3/1(reset3)
  [reset] -> q1/1(reset1)
  [vreset] -> q2/2(vreset2)
  [vreset] -> q0/2(vreset0)
  [vreset] -> q3/2(vreset3)
  [vreset] -> q1/2(vreset1)
  q0/1(vx) -> [vx0]
  q0/2(vy) -> [vy0]
  q0/3(vz) -> [vz0]
  q2/3(vz) -> [vz2]
  q2/1(vx) -> [vx2]
  q2/2(vy) -> [vy2]
  q3/1(vx) -> [vx3]
  q3/2(vy) -> [vy3]
  q3/3(vz) -> [vz3]
  q1/1(vx) -> [vx1]
  q1/2(vy) -> [vy1]
  q1/3(vz) -> [vz1]
  [vx0] -> Multiport Switch1/2
  [vx1] -> Multiport Switch1/3
  [vx2] -> Multiport Switch1/4
  [vx3] -> Multiport Switch1/5
  [vy0] -> Multiport Switch2/2
  [vy1] -> Multiport Switch2/3
  [vy2] -> Multiport Switch2/4
  [vy3] -> Multiport Switch2/5
  [q] -> Multiport Switch1/1
  [q] -> Multiport Switch2/1
  [q] -> Multiport Switch3/1
  [vz0] -> Multiport Switch3/2
  [vz1] -> Multiport Switch3/3
  [vz2] -> Multiport Switch3/4
  [vz3] -> Multiport Switch3/5
  Multiport Switch3/1 -> Add3/3, Memory3/1
  Switch Case/1 -> [q0]
  Switch Case/2 -> [q1]
  Switch Case/3 -> [q2]
  Switch Case/4 -> [q3]
  [q0] -> q0/Action
  [q2] -> q2/Action
  [q3] -> q3/Action
  [q1] -> q1/Action
  [q] -> Switch Case/1
  az1/1 -> [az1]
  ay1/1 -> [ay1]
  ax1/1 -> [ax1]
  beta/1 -> [beta]
  [beta] -> q1/4(beta)
  [ax1] -> q1/5(ax1)
  [ay1] -> q1/6(ay1)
  [az1] -> q1/7(az1)
  az3/1 -> q3/5(az3)

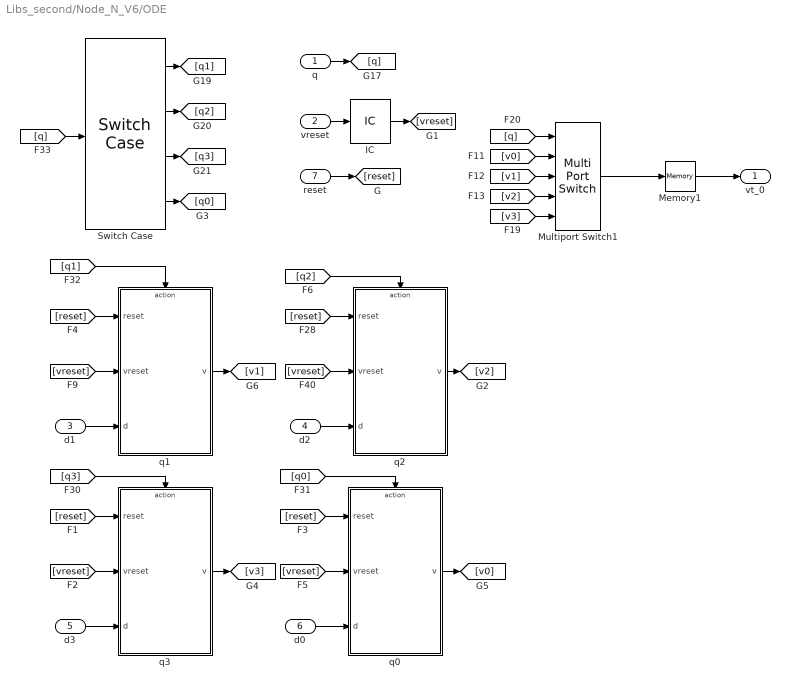
== system Libs_second/Node_N_V6/ODE ==
  q : Inport
  vreset : Inport  Port=2
  d1 : Inport  Port=3
  d2 : Inport  Port=4
  d3 : Inport  Port=5
  d0 : Inport  Port=6
  reset : Inport  Port=7
  IC : InitialCondition  Value=0
  Memory1 : Memory
  Multiport Switch1 : MultiPortSwitch  DataPortOrder=Zero-based contiguous  Inputs=4  zeroidx=on  SaturateOnIntegerOverflow=off  InputSameDT=off
  Switch Case : SwitchCase  CaseConditions={1,2,3,0}  ShowDefaultCase=off
  q0 : Subsystem  TreatAsAtomicUnit=on
  q1 : Subsystem  TreatAsAtomicUnit=on
  q2 : Subsystem  TreatAsAtomicUnit=on
  q3 : Subsystem  TreatAsAtomicUnit=on
  vt_0 : Outport
  wires:
  Multiport Switch1/1 -> Memory1/1
  IC/1 -> [vreset]
  vreset/1 -> IC/1
  reset/1 -> [reset]
  q/1 -> [q]
  q1/1(v) -> [v1]
  [q] -> Multiport Switch1/1
  [q] -> Switch Case/1
  [q1] -> q1/Action
  [reset] -> q1/1(reset)
  Switch Case/1 -> [q1]
  Switch Case/2 -> [q2]
  Switch Case/3 -> [q3]
  Switch Case/4 -> [q0]
  q2/1(v) -> [v2]
  d2/1 -> q2/3(d)
  [q2] -> q2/Action
  [vreset] -> q2/2(vreset)
  q3/1(v) -> [v3]
  d3/1 -> q3/3(d)
  [reset] -> q3/1(reset)
  [vreset] -> q3/2(vreset)
  q0/1(v) -> [v0]
  d0/1 -> q0/3(d)
  [reset] -> q0/1(reset)
  [vreset] -> q0/2(vreset)
  [q3] -> q3/Action
  [q0] -> q0/Action
  Memory1/1 -> vt_0/1
  [v0] -> Multiport Switch1/2
  [v1] -> Multiport Switch1/3
  [v2] -> Multiport Switch1/4
  [v3] -> Multiport Switch1/5
  [reset] -> q2/1(reset)
  [vreset] -> q1/2(vreset)
  d1/1 -> q1/3(d)

== system Libs_second/Node_M_V4/ODE/q0 ==
  reset0 : Inport
  vreset0 : Inport  Port=2
  ax0 : Inport  Port=3
  ay0 : Inport  Port=4
  az0 : Inport  Port=5
  Action Port : ActionPort  InitializeStates=reset
  Demux : Demux  Outputs=3
  Integrator1 : Integrator  ExternalReset=either  InitialConditionSource=external  InitialCondition=20
  Integrator2 : Integrator  ExternalReset=either  InitialConditionSource=external  InitialCondition=20
  Integrator3 : Integrator  ExternalReset=either  InitialConditionSource=external  InitialCondition=20
  ax0*vx : Product
  ay0*vy : Product
  az0*vz : Product
  vx : Outport
  vy : Outport  Port=2
  vz : Outport  Port=3
  wires:
  az0/1 -> az0*vz/2
  ay0/1 -> ay0*vy/2
  ax0/1 -> ax0*vx/2
  Demux/3 -> Integrator3/3
  Demux/2 -> Integrator2/3
  Demux/1 -> Integrator1/3
  vreset0/1 -> Demux/1
  az0*vz/1 -> Integrator3/1
  Integrator3/1 -> az0*vz/1, vz/1
  ay0*vy/1 -> Integrator2/1
  Integrator2/1 -> vy/1, ay0*vy/1
  Integrator1/1 -> vx/1, ax0*vx/1
  ax0*vx/1 -> Integrator1/1
  reset0/1 -> Integrator1/2, Integrator2/2, Integrator3/2

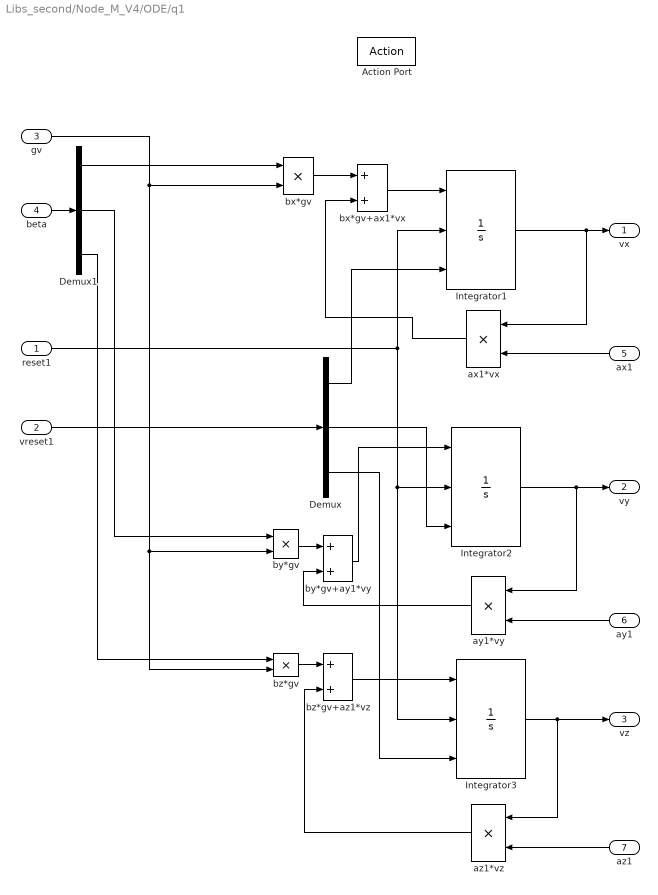
== system Libs_second/Node_M_V4/ODE/q1 ==
  reset1 : Inport
  vreset1 : Inport  Port=2
  gv : Inport  Port=3
  beta : Inport  Port=4
  ax1 : Inport  Port=5
  ay1 : Inport  Port=6
  az1 : Inport  Port=7
  Action Port : ActionPort  InitializeStates=reset
  Demux : Demux  Outputs=3
  Demux1 : Demux  Outputs=3
  Integrator1 : Integrator  ExternalReset=either  InitialConditionSource=external  InitialCondition=1
  Integrator2 : Integrator  ExternalReset=either  InitialConditionSource=external  InitialCondition=1
  Integrator3 : Integrator  ExternalReset=either  InitialConditionSource=external  InitialCondition=1
  ax1*vx : Product
  ay1*vy : Product
  az1*vz : Product
  bx*gv : Product
  bx*gv+ax1*vx : Sum
  by*gv : Product
  by*gv+ay1*vy : Sum
  bz*gv : Product
  bz*gv+az1*vz : Sum
  vx : Outport
  vy : Outport  Port=2
  vz : Outport  Port=3
  wires:
  Demux1/2 -> by*gv/1
  ax1*vx/1 -> bx*gv+ax1*vx/2
  bx*gv/1 -> bx*gv+ax1*vx/1
  ax1/1 -> ax1*vx/2
  bx*gv+ax1*vx/1 -> Integrator1/1
  by*gv+ay1*vy/1 -> Integrator2/1
  by*gv/1 -> by*gv+ay1*vy/1
  ay1*vy/1 -> by*gv+ay1*vy/2
  ay1/1 -> ay1*vy/2
  bz*gv+az1*vz/1 -> Integrator3/1
  az1*vz/1 -> bz*gv+az1*vz/2
  bz*gv/1 -> bz*gv+az1*vz/1
  az1/1 -> az1*vz/2
  Demux/3 -> Integrator3/3
  Demux/2 -> Integrator2/3
  Demux/1 -> Integrator1/3
  reset1/1 -> Integrator3/2, Integrator2/2, Integrator1/2
  gv/1 -> bz*gv/2, by*gv/2, bx*gv/2
  Integrator1/1 -> ax1*vx/1, vx/1
  Integrator2/1 -> vy/1, ay1*vy/1
  Integrator3/1 -> vz/1, az1*vz/1
  vreset1/1 -> Demux/1
  beta/1 -> Demux1/1
  Demux1/1 -> bx*gv/1
  Demux1/3 -> bz*gv/1

== system Libs_second/Node_M_V4/ODE/q2 ==
  reset2 : Inport
  vreset2 : Inport  Port=2
  ax2 : Inport  Port=3
  ay2 : Inport  Port=4
  az2 : Inport  Port=5
  Action Port : ActionPort  InitializeStates=reset
  Demux : Demux  Outputs=3
  Integrator1 : Integrator  ExternalReset=either  InitialConditionSource=external  InitialCondition=20
  Integrator2 : Integrator  ExternalReset=either  InitialConditionSource=external  InitialCondition=20
  Integrator3 : Integrator  ExternalReset=either  InitialConditionSource=external  InitialCondition=20
  ax2*vx : Product
  ay2*vy : Product
  az2*vz : Product
  vx : Outport
  vy : Outport  Port=2
  vz : Outport  Port=3
  wires:
  Demux/3 -> Integrator3/3
  Demux/2 -> Integrator2/3
  Demux/1 -> Integrator1/3
  vreset2/1 -> Demux/1
  az2*vz/1 -> Integrator3/1
  ay2*vy/1 -> Integrator2/1
  az2/1 -> az2*vz/2
  Integrator3/1 -> vz/1, az2*vz/1
  ay2/1 -> ay2*vy/2
  Integrator2/1 -> vy/1, ay2*vy/1
  Integrator1/1 -> vx/1, ax2*vx/1
  ax2/1 -> ax2*vx/2
  ax2*vx/1 -> Integrator1/1
  reset2/1 -> Integrator1/2, Integrator2/2, Integrator3/2

== system Libs_second/Node_M_V4/ODE/q3 ==
  reset3 : Inport
  vreset3 : Inport  Port=2
  ax3 : Inport  Port=3
  ay3 : Inport  Port=4
  az3 : Inport  Port=5
  ftheta : Inport  Port=6
  Action Port : ActionPort  InitializeStates=reset
  Demux : Demux  Outputs=3
  Integrator1 : Integrator  ExternalReset=either  InitialConditionSource=external  InitialCondition=133
  Integrator2 : Integrator  ExternalReset=either  InitialConditionSource=external  InitialCondition=133
  Integrator3 : Integrator  ExternalReset=either  InitialConditionSource=external  InitialCondition=133
  ax3*vx*lamda : Product  Inputs=3
  ay3*vy*lamda : Product  Inputs=3
  az3*vz* : Product
  vx : Outport
  vy : Outport  Port=2
  vz : Outport  Port=3
  wires:
  Demux/3 -> Integrator3/3
  Demux/2 -> Integrator2/3
  Demux/1 -> Integrator1/3
  vreset3/1 -> Demux/1
  az3*vz*/1 -> Integrator3/1
  az3/1 -> az3*vz*/2
  ay3/1 -> ay3*vy*lamda/3
  Integrator3/1 -> vz/1, az3*vz*/1
  Integrator2/1 -> vy/1, ay3*vy*lamda/1
  ay3*vy*lamda/1 -> Integrator2/1
  Integrator1/1 -> vx/1, ax3*vx*lamda/1
  ax3/1 -> ax3*vx*lamda/2
  ax3*vx*lamda/1 -> Integrator1/1
  reset3/1 -> Integrator1/2, Integrator2/2, Integrator3/2
  ftheta/1 -> ay3*vy*lamda/2, ax3*vx*lamda/3

== system Libs_second/Node_N_V6/ODE/q0 ==
  reset : Inport
  vreset : Inport  Port=2
  d : Inport  Port=3
  Action Port : ActionPort  InitializeStates=reset
  Integrator1 : Integrator  ExternalReset=either  InitialConditionSource=external  InitialCondition=20
  v : Outport
  wires:
  d/1 -> Integrator1/1
  vreset/1 -> Integrator1/3
  reset/1 -> Integrator1/2
  Integrator1/1 -> v/1

== system Libs_second/Node_N_V6/ODE/q1 ==
  reset : Inport
  vreset : Inport  Port=2
  d : Inport  Port=3
  Action Port : ActionPort  InitializeStates=reset
  Integrator1 : Integrator  ExternalReset=either  InitialConditionSource=external  InitialCondition=20
  v : Outport
  wires:
  vreset/1 -> Integrator1/3
  reset/1 -> Integrator1/2
  Integrator1/1 -> v/1
  d/1 -> Integrator1/1

== system Libs_second/Node_N_V6/ODE/q2 ==
  reset : Inport
  vreset : Inport  Port=2
  d : Inport  Port=3
  Action Port : ActionPort  InitializeStates=reset
  Integrator1 : Integrator  ExternalReset=either  InitialConditionSource=external  InitialCondition=20
  v : Outport
  wires:
  Integrator1/1 -> v/1
  reset/1 -> Integrator1/2
  vreset/1 -> Integrator1/3
  d/1 -> Integrator1/1

== system Libs_second/Node_N_V6/ODE/q3 ==
  reset : Inport
  vreset : Inport  Port=2
  d : Inport  Port=3
  Action Port : ActionPort  InitializeStates=reset
  Integrator1 : Integrator  ExternalReset=either  InitialConditionSource=external  InitialCondition=20
  v : Outport
  wires:
  d/1 -> Integrator1/1
  vreset/1 -> Integrator1/3
  reset/1 -> Integrator1/2
  Integrator1/1 -> v/1

== stateflow chart Libs_second/Node_M_V4/Automaton ==
  settings: executeAtInitialization=1
  state Resting_FR
    en: q=0;
    VT=VTin;
  state Stimulated
    en: q=1;
  state Plateau_ER
    en:q=3;
  state Upstroke
    en: q=2;
  (default) -> Resting_FR : {[ax0,ay0,az0,ax1,ay1,az1,ax2,ay2,az2,ax3,ay3,az3,bx1,by1,bz1]=pupdate;}
  Resting_FR -> Stimulated : [(gv>VT)&&v<=VT]{...
      | [ax0,ay0,az0,ax1,ay1,az1,ax2,ay2,az2,ax3,ay3,az3,bx1,by1,bz1]=pupdate;
      | VO_max=VO_maxin;
      | VR=VRin;
      | v_x_reset=v_x;
      | v_y_reset=v_y;
      | v_z_reset=v_z;
      | vno=v;VO=VO_max-80.1*sqrt(vno/VR);
      | [theta,ftheta]=vtheta(vno,VR,a,b,c,d,e);
      | reset;}
  Stimulated -> Resting_FR [order 2] : [(gv<=0)&&v<VT]{...
      | v_x_reset=v_x;
      | v_y_reset=v_y;
      | v_z_reset=v_z;
      | reset;}
  Stimulated -> Upstroke [order 1] : [v>=VT]{...
      | v_x_reset=(v_x-vx_d)*(VT-vt_d)/(v-vt_d)+vx_d;
      | v_y_reset=(v_y-vy_d)*(VT-vt_d)/(v-vt_d)+vy_d;
      | v_z_reset=(v_z-vz_d)*(VT-vt_d)/(v-vt_d)+vz_d;
      | reset;}
  Plateau_ER -> Resting_FR : [v<=VR]{...
      | v_x_reset=(v_x-vx_d)*(VR-vt_d)/(v-vt_d)+vx_d;
      | v_y_reset=(v_y-vy_d)*(VR-vt_d)/(v-vt_d)+vy_d;
      | v_z_reset=(v_z-vz_d)*(VR-vt_d)/(v-vt_d)+vz_d;
      | reset;}
  Upstroke -> Plateau_ER : [v>=VO]{...
      | v_x_reset=(v_x-vx_d)*(VO-vt_d)/(v-vt_d)+vx_d;
      | v_y_reset=(v_y-vy_d)*(VO-vt_d)/(v-vt_d)+vy_d;
      | v_z_reset=(v_z-vz_d)*(VO-vt_d)/(v-vt_d)+vz_d;
      | reset;}
  data: pax0 function_output double; pay0 function_output double; paz0 function_output double; pax1 function_output double; pay1 function_output double; paz1 function_output double; pax2 function_output double; pay2 function_output double; paz2 function_output double; pax3 function_output double; pay3 function_output double; paz3 function_output double; pbx1 function_output double; pby1 function_output double; pbz1 function_output double; vnin function_input double; VRi function_input double; ain function_input double; bin function_input double; cin function_input double; din function_input double; ein function_input double; thetaout function_output double; fthetatout function_output double; v input double; q output double; v_x input; v_y input; v_z input; v_x_reset output double =0; v_y_reset output double =0; v_z_reset output double =0; vno local double; VTin input; VRin input; VO_maxin input double; gv input; theta output double; ftheta output double; a input double; b input double; c input double; d input double; e input double; vt_d input double; vx_d input double; vy_d input double; vz_d input double; ax0 output; ay0 output; az0 output; ax1 output; ay1 output; az1 output; ax2 output; ay2 output; az2 output; ax3 output; ay3 output; az3 output; bx1 output; by1 output; bz1 output; ax0in input; ay0in input; az0in input; ax1in input; ay1in input; az1in input; ax2in input; ay2in input; az2in input; ax3in input; ay3in input; az3in input; bx1in input; by1in input; bz1in input; VO_max local; VR local; VT local; VO output double
  events: reset output EITHER_EDGE_EVENT
  function [pax0,pay0,paz0,pax1,pay1,paz1,pax2,pay2,paz2,pax3,pay3,paz3,pbx1,pby1,pbz1]=pupdate:
    | function [pax0,pay0,paz0,pax1,pay1,paz1,pax2,pay2,paz2,pax3,pay3,paz3,pbx1,pby1,pbz1]=pupdate
    | pax0=ax0in;
    | pay0=ay0in;
    | paz0=az0in;
    | pax1=ax1in;
    | pay1=ay1in;
    | paz1=az1in;
    | pax2=ax2in;
    | pay2=ay2in;
    | paz2=az2in;
    | pax3=ax3in;
    | pay3=ay3in;
    | paz3=az3in;
    | pbx1=bx1in;
    | pby1=by1in;
    | pbz1=bz1in;
  function [thetaout,fthetatout]  = vtheta(vnin,VRi,ain,bin,cin,din,ein):
    | function [thetaout,fthetatout]  = vtheta(vnin,VRi,ain,bin,cin,din,ein)
    | %Rate dependent factor
    | thetaout=vnin/VRi;
    | if thetaout<ein
    |     fthetatout=ain*exp(bin*thetaout)+cin*exp(-din*thetaout);
    | else
    |     fthetatout=ain*exp(bin*ein)+cin*exp(-din*ein);
    |     thetaout=ein;
    | end
    | 
    | end

== matlab function Libs_second/Node_NM_V4/ZeroPath ==
  data: pcfg output; dij input; dji input
function pcfg= Path(dij,dji)
%#codegen
CVi2j=1;
Dij=dij;
aij=1;
bij=0;
cij=0;

CVj2i=1;
Dji=dji;
aji=1;
bji=0;
cji=0;
C=5;

pcfg=[CVi2j,Dij, aij, bij, cij,CVj2i,Dji, aji,bji,cji,C];
end

== stateflow chart Libs_second/Sensing/Chart ==
  settings: executeAtInitialization=1
  state S
    state After_potential [parallel]
      settings: executionOrder=1
      state Timer
        du:
        t=temporalCount(msec);
        va=exp(-t)/RC;
      state Ini
      state waith
      waith -> S.After_potential.Timer : [pacing==0]
      (default) -> S.After_potential.Ini : /{t=0;va=0;}
      S.After_potential.Ini -> waith : [pacing>=1]
      S.After_potential.Timer -> waith : [pacing>=1]/{t=0;va=0;}
    state Pulse [parallel]
      settings: executionOrder=2
      state Ini
      state Timer
        du:
        t1=temporalCount(msec);
        v=amp;
      state waitl
      S.Pulse.Ini -> S.Pulse.Timer : [pacing>=1]
      (default) -> S.Pulse.Ini : /{t1=0;v=0;}
      waitl -> S.Pulse.Ini : [pacing==0]
      S.Pulse.Timer -> waitl : [after(3,msec)]/{v=0;}
  (default) -> S
  data: va output; t local; RC input; v output; t1 local; amp input; pacing input

== stateflow chart Libs_second/Sensing/Chart2 ==
  settings: executeAtInitialization=1
  state Ini
  Ini -> Ini [order 1] : clk[egm>=threshold]/{eve=1;}
  (default) -> Ini
  Ini -> Ini [order 2] : clk[egm<threshold]/{eve=0;}
  data: egm input; threshold input; eve output
  events: clk input RISING_EDGE_EVENT

== matlab function Libs_second/Sensing/Comba ==
  data: a input; y output; b input; c input; vadt input; vadr input; vvpa input
function y = aegm(a,b,c,vadt,vadr,vvpa)
%#codegen

y = a*(vadt-b*vadr+c*vvpa);

== matlab function Libs_second/Sensing/Combv ==
  data: d input; y1 output; b input; c1 input; e input; vvdt input; vvdr input; vvrt input; vvrr input; vapa input
function y1 = vegm(d,b,c1,e,vvdt,vvdr,vvrt,vvrr,vapa)
%#codegen

y1 = d*(vvdt-b*vvdr+e*(vvrt-b*vvrr)+c1*vapa);

== stateflow chart Libs_second/Electrode/Path2 ==
  state EGM1
    state De_wave_i [parallel]
      settings: executionOrder=1
      state Idle
        en:
        egm_d_i=[0 0 0 0]; wave_xi=0; wave_yi=0;
      state Active
        du:
        [egm_d_i,wave_xi,wave_yi]  = EGM(cvi,xi,yi,xj,yj,ti,Leads,C);
      EGM1.De_wave_i.Idle -> EGM1.De_wave_i.Active : [ti~=0]
      (default) -> EGM1.De_wave_i.Idle
      EGM1.De_wave_i.Active -> EGM1.De_wave_i.Idle : [ti==0]
    state De_wave_j [parallel]
      settings: executionOrder=2
      state Idle
        en:
        egm_d_j=[0 0 0 0]; wave_xj=0; wave_yj=0;
      state Active
        du:
        [egm_d_j,wave_xj,wave_yj]  = EGM(cvj,xj,yj,xi,yi,tj,Leads,C);
      EGM1.De_wave_j.Idle -> EGM1.De_wave_j.Active : [tj~=0]
      (default) -> EGM1.De_wave_j.Idle
      EGM1.De_wave_j.Active -> EGM1.De_wave_j.Idle : [tj==0]
    state Re_wave_i [parallel]
      settings: executionOrder=3
      state Idle
        en:
        egm_r_i=[0 0 0 0]; wave_xir=0; wave_yir=0;
      state Active
        du:
        [egm_r_i,wave_xir,wave_yir]  = EGM(cvi,xi,yi,xj,yj,tir,Leads,C);
      EGM1.Re_wave_i.Idle -> EGM1.Re_wave_i.Active : [tir~=0]
      (default) -> EGM1.Re_wave_i.Idle
      EGM1.Re_wave_i.Active -> EGM1.Re_wave_i.Idle : [tir==0]
    state Re_wave_j [parallel]
      settings: executionOrder=4
      state Idle
        en:
        egm_r_j=[0 0 0 0]; wave_xjr=0; wave_yjr=0;
      state Active
        du:
        [egm_r_j,wave_xjr,wave_yjr]  = EGM(cvj,xj,yj,xi,yi,tjr,Leads,C);
      EGM1.Re_wave_j.Idle -> EGM1.Re_wave_j.Active : [tjr~=0]
      (default) -> EGM1.Re_wave_j.Idle
      EGM1.Re_wave_j.Active -> EGM1.Re_wave_j.Idle : [tjr==0]
  (default) -> EGM1
  data: cv1in function_input; x1in function_input; y1in function_input; x2in function_input; y2in function_input; t1in function_input; electrodein function_input; Cin function_input; Potential_d function_output; x11 function_output; y11 function_output; xi input; yi input; xj input; yj input; cvi input; cvj input; ti input; tj input; tir input; tjr input; C input; egm_d_i output; egm_d_j output; egm_r_i output; egm_r_j output; wave_xi output; wave_yi output; wave_xj output; wave_yj output; Leads input; wave_xir output; wave_yir output; wave_xjr output; wave_yjr output
  function [Potential_d,x11,y11]  = EGM(cv1in,x1in,y1in,x2in,y2in,t1in,electrodein,Cin):
    | function [Potential_d,x11,y11]  = EGM(cv1in,x1in,y1in,x2in,y2in,t1in,electrodein,Cin)
    |     %#codegen
    |     % % The distance (mm) between the electrodes and the activation in z
    |     % direction
    |     % Compute theta2: the angle between (x1,y1)-->(x2,y2) and x axis;
    |     cos_theta2=(x2in-x1in)/sqrt((x2in-x1in)^2+(y2in-y1in)^2);
    |     sin_theta2=(y1in-y2in)/sqrt((x2in-x1in)^2+(y2in-y1in)^2);
    |     if cos_theta2~=0
    |     tan_theta2=(y1in-y2in)/(x2in-x1in);
    |     else
    |      tan_theta2=0;   
    |     end
    |     
    |     N=length(electrodein)-4; % The number of (x,y,z) of total micro electrodes;
    |     
    |     vtip=electrodein(length(electrodein)); % The number of micro electrodes of the ventricular tip part;
    |     vring=electrodein(length(electrodein)-1); % The number of micro electrodes of the ventricular ring part;
    |     atip=electrodein(length(electrodein)-2); % The number of micro electrodes of the atrial tip part;
    |     aring=electrodein(length(electrodein)-3); % The number of micro electrodes of the atrial ring part;
    |     Potential_d=zeros(1,4); % To store the EGM sensed by atrial ring, tip, ventricular ring and tip part;
    |     p=zeros(1,N/3); % To store the signals sensed by all the micro electrodes;
    | 
    |     L=1; % weighting factor of the longitudinal dipole
    |     T=0.1; % weighting factor of the transversal dipole
    |     % Only when the path is active, can the cells contribute to the EGM
    |     m=0;
    |     for j=1:3:(N-2)
    |         % The location of the micro electrode
    |         x3=electrodein(j);
    |         y3=electrodein(j+1);
    |         zin=electrodein(j+2);
    |         % The closest point to the micro electrode
    |         if cos_theta2~=0
    |         y4=(y2in+tan_theta2*(x2in-x3+tan_theta2*y3))/(1+tan_theta2^2);
    |         x4=tan_theta2*y4-tan_theta2*y3+x3;
    |         else
    |             y4=y3;
    |             x4=x1in;
    |         end
    |         d=sqrt((x3-x4)^2+(y3-y4)^2+zin^2);
    |         
    |         x11=x1in+cv1in*t1in*cos_theta2; % the dipole position
    |         y11=y1in-cv1in*t1in*sin_theta2;
    |         % Compute theta1: the angle between (x11,y11)-->(x3,y3) and x axis;
    |         if x3==x11 && y3==y11
    |          cos_theta1=0;
    |          sin_theta1=0;
    |         else
    |         cos_theta1=(x3-x11)/sqrt((x3-x11)^2+(y3-y11)^2);
    |         sin_theta1=(y3-y11)/sqrt((x3-x11)^2+(y3-y11)^2);
    |         end
    |         % alfa=theta1+theta2, the angle between (x11,y11)-->(x3,y3) and (x11,y11)-->(x2,y2)
    |         cos_alfa = cos_theta1*cos_theta2 - sin_theta1*sin_theta2;
    |         
    |         h1=sqrt((x4-x11)^2+(y4-y11)^2)*sign(cos_alfa); % the distance between the dipole and (x4,y4), when the dipole is approaching, h1>0;
    |         r1=sqrt((d^2+h1^2)); % the distance between the dipole and the micro electrode;
    |         EGML1=L*h1/(r1^3);
    |         EGMT1=(-1)*T*d/(r1^3);
    |         EGMall=EGML1+EGMT1;
    |         m=m+1;
    |         p(m) =EGMall*Cin;
    |     end
    |     s=1;
    |     e=aring;
    |     Potential_d(1)=sum(p(s:e));
    |     s=e+1;
    |     e=s+atip-1;
    |     Potential_d(2)=sum(p(s:e));
    |     s=e+1;
    |     e=s+vring-1;
    |     Potential_d(3)=sum(p(s:e));
    |     s=e+1;
    |     e=s+vtip-1;
    |     Potential_d(4)=sum(p(s:e));
    | 
    | end

== stateflow chart Libs_second/Sensing/Chart1 ==
  settings: executeAtInitialization=1
  state Ini
  Ini -> Ini [order 1] : clk[egm>=threshold]/{eve=1;}
  (default) -> Ini
  Ini -> Ini [order 2] : clk[egm<threshold]/{eve=0;}
  data: egm input; threshold input; eve output
  events: clk input RISING_EDGE_EVENT

== stateflow chart Libs_second/Sensing/Chart3 ==
  settings: executeAtInitialization=1
  state S
    state After_potential [parallel]
      settings: executionOrder=1
      state Timer
        du:
        t=temporalCount(msec);
        va=exp(-t)/RC;
      state Ini
      state waith
      waith -> S.After_potential.Timer : [pacing==0]
      (default) -> S.After_potential.Ini : /{t=0;va=0;}
      S.After_potential.Ini -> waith : [pacing>=1]
      S.After_potential.Timer -> waith : [pacing>=1]/{t=0;va=0;}
    state Pulse [parallel]
      settings: executionOrder=2
      state Ini
      state Timer
        du:
        t1=temporalCount(msec);
        v=amp;
      state waitl
      S.Pulse.Ini -> S.Pulse.Timer : [pacing>=1]
      (default) -> S.Pulse.Ini : /{t1=0;v=0;}
      waitl -> S.Pulse.Ini : [pacing==0]
      S.Pulse.Timer -> waitl : [after(3,msec)]/{v=0;}
  (default) -> S
  data: va output; t local; RC input; v output; t1 local; amp input; pacing input
